simulink model "r2_b16a4x512f"  (R2012b)
settings: Solver=VariableStepDiscrete  SolverMode=SingleTasking  StartTime=0.0  StopTime=1  RelTol=1e-3
undefined symbols (not defined in the file): fft_stages, n_bits_ants, n_bits_xengs
libraries: xbsIndex_r4 x27410, casper_library_misc x230, xbsReplacements_r4 x24, casper_library_delays x8, xps_library x5, casper_library_communications x4
(part 116 of 229)

== system r2_b16a4x512f/sys2/xeng/baseline_tap7/dual_pol_cmac ==
  a1 : Inport
  a2 : Inport  Port=2
  acc_in : Inport  Port=3
  sync : Inport  Port=4
  valid_in : Inport  Port=5
  Concat : xbsIndex_r4/Concat  num_inputs=4  dbl_ovrd=off  block_type=concat
      settings: block_version=9.2.01
  Constant1 : xbsIndex_r4/Constant  const=0  gui_display_data_type=Fixed-point  arith_type=Unsigned  n_bits=1  bin_pt=0  preci_type=Single  exp_width=8  frac_width=24  explicit_period=on  period=1  equ=P=C  opselect=C  inp2=PCIN>>17  opr=+  inp1=P  carry=CIN  dbl_ovrd=off  block_type=constant
      settings: block_version=9.2.01
  Constant2 : xbsIndex_r4/Constant  const=0  gui_display_data_type=Fixed-point  arith_type=Unsigned  n_bits=1  bin_pt=0  preci_type=Single  exp_width=8  frac_width=24  explicit_period=on  period=1  equ=P=C  opselect=C  inp2=PCIN>>17  opr=+  inp1=P  carry=CIN  dbl_ovrd=off  block_type=constant
      settings: block_version=9.2.01
  Constant4 : xbsIndex_r4/Constant  const=0  gui_display_data_type=Fixed-point  arith_type=Unsigned  n_bits=1  bin_pt=0  preci_type=Single  exp_width=8  frac_width=24  explicit_period=on  period=1  equ=P=C  opselect=C  inp2=PCIN>>17  opr=+  inp1=P  carry=CIN  dbl_ovrd=off  block_type=constant
      settings: block_version=9.2.01
  Slice{,1,6,10} (4 alike) : xbsIndex_r4/Slice  nbits=2*n_bits  boolean_output=off  mode=Upper Bit Location + Width  bit1=0  base1=MSB of Input  bit0=0  base0=LSB of Input  dbl_ovrd=off  block_type=slice
      Slice settings: infoedit="Extracts a given range of bits from each input sample and presents it at the output.  The output type is ordinarily unsigned with binary point at zero, but can be Boolean when the slice is one bit wide.<P><P>Hardware notes: In hardware this block costs nothing."  block_version=9.2.01
      Slice1 settings: infoedit="Extracts a given range of bits from each input sample and presents it at the output.  The output type is ordinarily unsigned with binary point at zero, but can be Boolean when the slice is one bit wide.<P><P>Hardware notes: In hardware this block costs nothing."  block_version=9.2.01
      Slice10 settings: block_version=9.2.01
      Slice6 settings: infoedit="Extracts a given range of bits from each input sample and presents it at the output.  The output type is ordinarily unsigned with binary point at zero, but can be Boolean when the slice is one bit wide.<P><P>Hardware notes: In hardware this block costs nothing."  block_version=9.2.01
  Slice11 : xbsIndex_r4/Slice  nbits=2*n_bits_out  boolean_output=off  mode=Upper Bit Location + Width  bit1=-6*n_bits_out  base1=MSB of Input  bit0=0  base0=LSB of Input  dbl_ovrd=off  block_type=slice
      settings: infoedit="Extracts a given range of bits from each input sample and presents it at the output.  The output type is ordinarily unsigned with binary point at zero, but can be Boolean when the slice is one bit wide.<P><P>Hardware notes: In hardware this block costs nothing."  block_version=9.2.01
  Slice2 : xbsIndex_r4/Slice  nbits=2*n_bits_out  boolean_output=off  mode=Upper Bit Location + Width  bit1=0  base1=MSB of Input  bit0=0  base0=LSB of Input  dbl_ovrd=off  block_type=slice
      settings: infoedit="Extracts a given range of bits from each input sample and presents it at the output.  The output type is ordinarily unsigned with binary point at zero, but can be Boolean when the slice is one bit wide.<P><P>Hardware notes: In hardware this block costs nothing."  block_version=9.2.01
  Slice{3..4,7,9} (4 alike) : xbsIndex_r4/Slice  nbits=2*n_bits  boolean_output=off  mode=Upper Bit Location + Width  bit1=-2*n_bits  base1=MSB of Input  bit0=0  base0=LSB of Input  dbl_ovrd=off  block_type=slice
      Slice3 settings: infoedit="Extracts a given range of bits from each input sample and presents it at the output.  The output type is ordinarily unsigned with binary point at zero, but can be Boolean when the slice is one bit wide.<P><P>Hardware notes: In hardware this block costs nothing."  block_version=9.2.01
      Slice4 settings: infoedit="Extracts a given range of bits from each input sample and presents it at the output.  The output type is ordinarily unsigned with binary point at zero, but can be Boolean when the slice is one bit wide.<P><P>Hardware notes: In hardware this block costs nothing."  block_version=9.2.01
      Slice7 settings: infoedit="Extracts a given range of bits from each input sample and presents it at the output.  The output type is ordinarily unsigned with binary point at zero, but can be Boolean when the slice is one bit wide.<P><P>Hardware notes: In hardware this block costs nothing."  block_version=9.2.01
      Slice9 settings: block_version=9.2.01
  Slice5 : xbsIndex_r4/Slice  nbits=2*n_bits_out  boolean_output=off  mode=Upper Bit Location + Width  bit1=-2*n_bits_out  base1=MSB of Input  bit0=0  base0=LSB of Input  dbl_ovrd=off  block_type=slice
      settings: infoedit="Extracts a given range of bits from each input sample and presents it at the output.  The output type is ordinarily unsigned with binary point at zero, but can be Boolean when the slice is one bit wide.<P><P>Hardware notes: In hardware this block costs nothing."  block_version=9.2.01
  Slice8 : xbsIndex_r4/Slice  nbits=2*n_bits_out  boolean_output=off  mode=Upper Bit Location + Width  bit1=-4*n_bits_out  base1=MSB of Input  bit0=0  base0=LSB of Input  dbl_ovrd=off  block_type=slice
      settings: infoedit="Extracts a given range of bits from each input sample and presents it at the output.  The output type is ordinarily unsigned with binary point at zero, but can be Boolean when the slice is one bit wide.<P><P>Hardware notes: In hardware this block costs nothing."  block_version=9.2.01
  Terminator : Terminator
  Terminator1 : Terminator
  Terminator2 : Terminator
  cmac1 : Subsystem  Tag=cmac  AncestorBlock=casper_library_correlator/cmac  mask(cmac){acc_len=256, n_bits_a=8, bin_pt_a=7, n_bits_b=8, bin_pt_b=7, quantization=Truncate, overflow=Wrap, mult_latency=4, add_latency=3, in_latency=0, conv_latency=0, multiplier_implementation=embedded multiplier core}
      mask prompts: acc_len "Number of Accumulations"; n_bits_a "Number of bits 'a'"; bin_pt_a "Binary point 'a'"; n_bits_b "Number of bits 'b'"; bin_pt_b "Binary point 'b'"; quantization "Quantisation"; mult_latency "Multiplier Latency"; add_latency "Adder Latency"; in_latency "Input Latency"; conv_latency "Convert Latency"; multiplier_implementation "Multiplier Implementation"
      mask help: A complex multiply-accumulate block. Full precision.
      mask init: same as r2_b16a4x512f/sys0/xeng/auto_tap/dual_pol_cmac/cmac1
      mask TypeOptions quantization: Truncate | Round  (unbiased: +/- Inf) | Round  (unbiased: Even Values)
      mask TypeOptions overflow: Wrap | Saturate | Flag as error
      mask TypeOptions multiplier_implementation: behavioral HDL | standard core | embedded multiplier core
  cmac2 : Subsystem  Tag=cmac  AncestorBlock=casper_library_correlator/cmac  mask(cmac){acc_len=256, n_bits_a=8, bin_pt_a=7, n_bits_b=8, bin_pt_b=7, quantization=Truncate, overflow=Wrap, mult_latency=4, add_latency=3, in_latency=0, conv_latency=0, multiplier_implementation=embedded multiplier core}
      mask prompts: acc_len "Number of Accumulations"; n_bits_a "Number of bits 'a'"; bin_pt_a "Binary point 'a'"; n_bits_b "Number of bits 'b'"; bin_pt_b "Binary point 'b'"; quantization "Quantisation"; mult_latency "Multiplier Latency"; add_latency "Adder Latency"; in_latency "Input Latency"; conv_latency "Convert Latency"; multiplier_implementation "Multiplier Implementation"
      mask help: A complex multiply-accumulate block. Full precision.
      mask init: same as r2_b16a4x512f/sys0/xeng/auto_tap/dual_pol_cmac/cmac1
      mask TypeOptions quantization: Truncate | Round  (unbiased: +/- Inf) | Round  (unbiased: Even Values)
      mask TypeOptions overflow: Wrap | Saturate | Flag as error
      mask TypeOptions multiplier_implementation: behavioral HDL | standard core | embedded multiplier core
  cmac3 : Subsystem  Tag=cmac  AncestorBlock=casper_library_correlator/cmac  mask(cmac){acc_len=256, n_bits_a=8, bin_pt_a=7, n_bits_b=8, bin_pt_b=7, quantization=Truncate, overflow=Wrap, mult_latency=4, add_latency=3, in_latency=0, conv_latency=0, multiplier_implementation=embedded multiplier core}
      mask prompts: acc_len "Number of Accumulations"; n_bits_a "Number of bits 'a'"; bin_pt_a "Binary point 'a'"; n_bits_b "Number of bits 'b'"; bin_pt_b "Binary point 'b'"; quantization "Quantisation"; mult_latency "Multiplier Latency"; add_latency "Adder Latency"; in_latency "Input Latency"; conv_latency "Convert Latency"; multiplier_implementation "Multiplier Implementation"
      mask help: A complex multiply-accumulate block. Full precision.
      mask init: same as r2_b16a4x512f/sys0/xeng/auto_tap/dual_pol_cmac/cmac1
      mask TypeOptions quantization: Truncate | Round  (unbiased: +/- Inf) | Round  (unbiased: Even Values)
      mask TypeOptions overflow: Wrap | Saturate | Flag as error
      mask TypeOptions multiplier_implementation: behavioral HDL | standard core | embedded multiplier core
  cmac4 : Subsystem  Tag=cmac  AncestorBlock=casper_library_correlator/cmac  mask(cmac){acc_len=256, n_bits_a=8, bin_pt_a=7, n_bits_b=8, bin_pt_b=7, quantization=Truncate, overflow=Wrap, mult_latency=4, add_latency=3, in_latency=0, conv_latency=0, multiplier_implementation=embedded multiplier core}
      mask prompts: acc_len "Number of Accumulations"; n_bits_a "Number of bits 'a'"; bin_pt_a "Binary point 'a'"; n_bits_b "Number of bits 'b'"; bin_pt_b "Binary point 'b'"; quantization "Quantisation"; mult_latency "Multiplier Latency"; add_latency "Adder Latency"; in_latency "Input Latency"; conv_latency "Convert Latency"; multiplier_implementation "Multiplier Implementation"
      mask help: A complex multiply-accumulate block. Full precision.
      mask init: same as r2_b16a4x512f/sys0/xeng/auto_tap/dual_pol_cmac/cmac1
      mask TypeOptions quantization: Truncate | Round  (unbiased: +/- Inf) | Round  (unbiased: Even Values)
      mask TypeOptions overflow: Wrap | Saturate | Flag as error
      mask TypeOptions multiplier_implementation: behavioral HDL | standard core | embedded multiplier core
  acc_out : Outport
  valid_out : Outport  Port=2
  wires:
  acc_in/1 -> Slice2/1, Slice5/1, Slice8/1, Slice11/1
  a2/1 -> Slice10/1, Slice7/1, Slice4/1, Slice1/1
  a1/1 -> Slice9/1, Slice6/1, Slice3/1, Slice/1
  cmac4/1(acc_out) -> Concat/4
  cmac3/1(acc_out) -> Concat/3
  cmac2/1(acc_out) -> Concat/2
  cmac1/1(acc_out) -> Concat/1
  cmac4/2(valid_out) -> valid_out/1
  cmac3/2(valid_out) -> Terminator2/1
  cmac2/2(valid_out) -> Terminator1/1
  sync/1 -> cmac4/4(sync), cmac3/4(sync), cmac2/4(sync), cmac1/4(sync)
  Slice11/1 -> cmac4/3(acc_in)
  Slice10/1 -> cmac4/2(c+di)
  Slice9/1 -> cmac4/1(a+bi)
  Constant4/1 -> cmac3/5(valid_in)
  Slice8/1 -> cmac3/3(acc_in)
  Slice7/1 -> cmac3/2(c+di)
  Slice6/1 -> cmac3/1(a+bi)
  Constant1/1 -> cmac2/5(valid_in)
  cmac1/2(valid_out) -> Terminator/1
  valid_in/1 -> cmac4/5(valid_in)
  Concat/1 -> acc_out/1
  Slice5/1 -> cmac2/3(acc_in)
  Slice4/1 -> cmac2/2(c+di)
  Slice3/1 -> cmac2/1(a+bi)
  Slice2/1 -> cmac1/3(acc_in)
  Slice1/1 -> cmac1/2(c+di)
  Slice/1 -> cmac1/1(a+bi)
  Constant2/1 -> cmac1/5(valid_in)

== system r2_b16a4x512f/sys2/xeng/baseline_tap8/delay ==
  din : Inport
  constant : xbsIndex_r4/Constant  const=1  gui_display_data_type=Fixed-point  arith_type=Boolean  n_bits=16  bin_pt=14  preci_type=Single  exp_width=8  frac_width=24  explicit_period=on  period=1  equ=P=C  opselect=C  inp2=PCIN>>17  opr=+  inp1=P  carry=CIN  dbl_ovrd=off  block_type=constant
  counter : xbsIndex_r4/Counter  cnt_type=Count Limited  cnt_to=DelayLen - bram_latency - 1  operation=Up  start_count=0  cnt_by_val=1  arith_type=Unsigned  n_bits=8  bin_pt=0  load_pin=off  rst=off  en=off  explicit_period=on  period=1  dbl_ovrd=off  use_behavioral_HDL=off  implementation=Fabric  use_rpm=off  block_type=counter
  ram : xbsIndex_r4/Single Port RAM  depth=256  initVector=0  distributed_mem=Block RAM  write_mode=Read Before Write  rst=off  init_reg=0  en=off  latency=bram_latency  dbl_ovrd=off  optimize=Area  block_type=spram
  dout : Outport
  wires:
  counter/1 -> ram/1
  din/1 -> ram/2
  constant/1 -> ram/3
  ram/1 -> dout/1

== system r2_b16a4x512f/sys2/xeng/baseline_tap8/dual_pol_cmac ==
  a1 : Inport
  a2 : Inport  Port=2
  acc_in : Inport  Port=3
  sync : Inport  Port=4
  valid_in : Inport  Port=5
  Concat : xbsIndex_r4/Concat  num_inputs=4  dbl_ovrd=off  block_type=concat
      settings: block_version=9.2.01
  Constant1 : xbsIndex_r4/Constant  const=0  gui_display_data_type=Fixed-point  arith_type=Unsigned  n_bits=1  bin_pt=0  preci_type=Single  exp_width=8  frac_width=24  explicit_period=on  period=1  equ=P=C  opselect=C  inp2=PCIN>>17  opr=+  inp1=P  carry=CIN  dbl_ovrd=off  block_type=constant
      settings: block_version=9.2.01
  Constant2 : xbsIndex_r4/Constant  const=0  gui_display_data_type=Fixed-point  arith_type=Unsigned  n_bits=1  bin_pt=0  preci_type=Single  exp_width=8  frac_width=24  explicit_period=on  period=1  equ=P=C  opselect=C  inp2=PCIN>>17  opr=+  inp1=P  carry=CIN  dbl_ovrd=off  block_type=constant
      settings: block_version=9.2.01
  Constant4 : xbsIndex_r4/Constant  const=0  gui_display_data_type=Fixed-point  arith_type=Unsigned  n_bits=1  bin_pt=0  preci_type=Single  exp_width=8  frac_width=24  explicit_period=on  period=1  equ=P=C  opselect=C  inp2=PCIN>>17  opr=+  inp1=P  carry=CIN  dbl_ovrd=off  block_type=constant
      settings: block_version=9.2.01
  Slice{,1,6,10} (4 alike) : xbsIndex_r4/Slice  nbits=2*n_bits  boolean_output=off  mode=Upper Bit Location + Width  bit1=0  base1=MSB of Input  bit0=0  base0=LSB of Input  dbl_ovrd=off  block_type=slice
      Slice settings: infoedit="Extracts a given range of bits from each input sample and presents it at the output.  The output type is ordinarily unsigned with binary point at zero, but can be Boolean when the slice is one bit wide.<P><P>Hardware notes: In hardware this block costs nothing."  block_version=9.2.01
      Slice1 settings: infoedit="Extracts a given range of bits from each input sample and presents it at the output.  The output type is ordinarily unsigned with binary point at zero, but can be Boolean when the slice is one bit wide.<P><P>Hardware notes: In hardware this block costs nothing."  block_version=9.2.01
      Slice10 settings: block_version=9.2.01
      Slice6 settings: infoedit="Extracts a given range of bits from each input sample and presents it at the output.  The output type is ordinarily unsigned with binary point at zero, but can be Boolean when the slice is one bit wide.<P><P>Hardware notes: In hardware this block costs nothing."  block_version=9.2.01
  Slice11 : xbsIndex_r4/Slice  nbits=2*n_bits_out  boolean_output=off  mode=Upper Bit Location + Width  bit1=-6*n_bits_out  base1=MSB of Input  bit0=0  base0=LSB of Input  dbl_ovrd=off  block_type=slice
      settings: infoedit="Extracts a given range of bits from each input sample and presents it at the output.  The output type is ordinarily unsigned with binary point at zero, but can be Boolean when the slice is one bit wide.<P><P>Hardware notes: In hardware this block costs nothing."  block_version=9.2.01
  Slice2 : xbsIndex_r4/Slice  nbits=2*n_bits_out  boolean_output=off  mode=Upper Bit Location + Width  bit1=0  base1=MSB of Input  bit0=0  base0=LSB of Input  dbl_ovrd=off  block_type=slice
      settings: infoedit="Extracts a given range of bits from each input sample and presents it at the output.  The output type is ordinarily unsigned with binary point at zero, but can be Boolean when the slice is one bit wide.<P><P>Hardware notes: In hardware this block costs nothing."  block_version=9.2.01
  Slice{3..4,7,9} (4 alike) : xbsIndex_r4/Slice  nbits=2*n_bits  boolean_output=off  mode=Upper Bit Location + Width  bit1=-2*n_bits  base1=MSB of Input  bit0=0  base0=LSB of Input  dbl_ovrd=off  block_type=slice
      Slice3 settings: infoedit="Extracts a given range of bits from each input sample and presents it at the output.  The output type is ordinarily unsigned with binary point at zero, but can be Boolean when the slice is one bit wide.<P><P>Hardware notes: In hardware this block costs nothing."  block_version=9.2.01
      Slice4 settings: infoedit="Extracts a given range of bits from each input sample and presents it at the output.  The output type is ordinarily unsigned with binary point at zero, but can be Boolean when the slice is one bit wide.<P><P>Hardware notes: In hardware this block costs nothing."  block_version=9.2.01
      Slice7 settings: infoedit="Extracts a given range of bits from each input sample and presents it at the output.  The output type is ordinarily unsigned with binary point at zero, but can be Boolean when the slice is one bit wide.<P><P>Hardware notes: In hardware this block costs nothing."  block_version=9.2.01
      Slice9 settings: block_version=9.2.01
  Slice5 : xbsIndex_r4/Slice  nbits=2*n_bits_out  boolean_output=off  mode=Upper Bit Location + Width  bit1=-2*n_bits_out  base1=MSB of Input  bit0=0  base0=LSB of Input  dbl_ovrd=off  block_type=slice
      settings: infoedit="Extracts a given range of bits from each input sample and presents it at the output.  The output type is ordinarily unsigned with binary point at zero, but can be Boolean when the slice is one bit wide.<P><P>Hardware notes: In hardware this block costs nothing."  block_version=9.2.01
  Slice8 : xbsIndex_r4/Slice  nbits=2*n_bits_out  boolean_output=off  mode=Upper Bit Location + Width  bit1=-4*n_bits_out  base1=MSB of Input  bit0=0  base0=LSB of Input  dbl_ovrd=off  block_type=slice
      settings: infoedit="Extracts a given range of bits from each input sample and presents it at the output.  The output type is ordinarily unsigned with binary point at zero, but can be Boolean when the slice is one bit wide.<P><P>Hardware notes: In hardware this block costs nothing."  block_version=9.2.01
  Terminator : Terminator
  Terminator1 : Terminator
  Terminator2 : Terminator
  cmac1 : Subsystem  Tag=cmac  AncestorBlock=casper_library_correlator/cmac  mask(cmac){acc_len=256, n_bits_a=8, bin_pt_a=7, n_bits_b=8, bin_pt_b=7, quantization=Truncate, overflow=Wrap, mult_latency=4, add_latency=3, in_latency=0, conv_latency=0, multiplier_implementation=embedded multiplier core}
      mask prompts: acc_len "Number of Accumulations"; n_bits_a "Number of bits 'a'"; bin_pt_a "Binary point 'a'"; n_bits_b "Number of bits 'b'"; bin_pt_b "Binary point 'b'"; quantization "Quantisation"; mult_latency "Multiplier Latency"; add_latency "Adder Latency"; in_latency "Input Latency"; conv_latency "Convert Latency"; multiplier_implementation "Multiplier Implementation"
      mask help: A complex multiply-accumulate block. Full precision.
      mask init: same as r2_b16a4x512f/sys0/xeng/auto_tap/dual_pol_cmac/cmac1
      mask TypeOptions quantization: Truncate | Round  (unbiased: +/- Inf) | Round  (unbiased: Even Values)
      mask TypeOptions overflow: Wrap | Saturate | Flag as error
      mask TypeOptions multiplier_implementation: behavioral HDL | standard core | embedded multiplier core
  cmac2 : Subsystem  Tag=cmac  AncestorBlock=casper_library_correlator/cmac  mask(cmac){acc_len=256, n_bits_a=8, bin_pt_a=7, n_bits_b=8, bin_pt_b=7, quantization=Truncate, overflow=Wrap, mult_latency=4, add_latency=3, in_latency=0, conv_latency=0, multiplier_implementation=embedded multiplier core}
      mask prompts: acc_len "Number of Accumulations"; n_bits_a "Number of bits 'a'"; bin_pt_a "Binary point 'a'"; n_bits_b "Number of bits 'b'"; bin_pt_b "Binary point 'b'"; quantization "Quantisation"; mult_latency "Multiplier Latency"; add_latency "Adder Latency"; in_latency "Input Latency"; conv_latency "Convert Latency"; multiplier_implementation "Multiplier Implementation"
      mask help: A complex multiply-accumulate block. Full precision.
      mask init: same as r2_b16a4x512f/sys0/xeng/auto_tap/dual_pol_cmac/cmac1
      mask TypeOptions quantization: Truncate | Round  (unbiased: +/- Inf) | Round  (unbiased: Even Values)
      mask TypeOptions overflow: Wrap | Saturate | Flag as error
      mask TypeOptions multiplier_implementation: behavioral HDL | standard core | embedded multiplier core
  cmac3 : Subsystem  Tag=cmac  AncestorBlock=casper_library_correlator/cmac  mask(cmac){acc_len=256, n_bits_a=8, bin_pt_a=7, n_bits_b=8, bin_pt_b=7, quantization=Truncate, overflow=Wrap, mult_latency=4, add_latency=3, in_latency=0, conv_latency=0, multiplier_implementation=embedded multiplier core}
      mask prompts: acc_len "Number of Accumulations"; n_bits_a "Number of bits 'a'"; bin_pt_a "Binary point 'a'"; n_bits_b "Number of bits 'b'"; bin_pt_b "Binary point 'b'"; quantization "Quantisation"; mult_latency "Multiplier Latency"; add_latency "Adder Latency"; in_latency "Input Latency"; conv_latency "Convert Latency"; multiplier_implementation "Multiplier Implementation"
      mask help: A complex multiply-accumulate block. Full precision.
      mask init: same as r2_b16a4x512f/sys0/xeng/auto_tap/dual_pol_cmac/cmac1
      mask TypeOptions quantization: Truncate | Round  (unbiased: +/- Inf) | Round  (unbiased: Even Values)
      mask TypeOptions overflow: Wrap | Saturate | Flag as error
      mask TypeOptions multiplier_implementation: behavioral HDL | standard core | embedded multiplier core
  cmac4 : Subsystem  Tag=cmac  AncestorBlock=casper_library_correlator/cmac  mask(cmac){acc_len=256, n_bits_a=8, bin_pt_a=7, n_bits_b=8, bin_pt_b=7, quantization=Truncate, overflow=Wrap, mult_latency=4, add_latency=3, in_latency=0, conv_latency=0, multiplier_implementation=embedded multiplier core}
      mask prompts: acc_len "Number of Accumulations"; n_bits_a "Number of bits 'a'"; bin_pt_a "Binary point 'a'"; n_bits_b "Number of bits 'b'"; bin_pt_b "Binary point 'b'"; quantization "Quantisation"; mult_latency "Multiplier Latency"; add_latency "Adder Latency"; in_latency "Input Latency"; conv_latency "Convert Latency"; multiplier_implementation "Multiplier Implementation"
      mask help: A complex multiply-accumulate block. Full precision.
      mask init: same as r2_b16a4x512f/sys0/xeng/auto_tap/dual_pol_cmac/cmac1
      mask TypeOptions quantization: Truncate | Round  (unbiased: +/- Inf) | Round  (unbiased: Even Values)
      mask TypeOptions overflow: Wrap | Saturate | Flag as error
      mask TypeOptions multiplier_implementation: behavioral HDL | standard core | embedded multiplier core
  acc_out : Outport
  valid_out : Outport  Port=2
  wires:
  acc_in/1 -> Slice2/1, Slice5/1, Slice8/1, Slice11/1
  a2/1 -> Slice10/1, Slice7/1, Slice4/1, Slice1/1
  a1/1 -> Slice9/1, Slice6/1, Slice3/1, Slice/1
  cmac4/1(acc_out) -> Concat/4
  cmac3/1(acc_out) -> Concat/3
  cmac2/1(acc_out) -> Concat/2
  cmac1/1(acc_out) -> Concat/1
  cmac4/2(valid_out) -> valid_out/1
  cmac3/2(valid_out) -> Terminator2/1
  cmac2/2(valid_out) -> Terminator1/1
  sync/1 -> cmac4/4(sync), cmac3/4(sync), cmac2/4(sync), cmac1/4(sync)
  Slice11/1 -> cmac4/3(acc_in)
  Slice10/1 -> cmac4/2(c+di)
  Slice9/1 -> cmac4/1(a+bi)
  Constant4/1 -> cmac3/5(valid_in)
  Slice8/1 -> cmac3/3(acc_in)
  Slice7/1 -> cmac3/2(c+di)
  Slice6/1 -> cmac3/1(a+bi)
  Constant1/1 -> cmac2/5(valid_in)
  cmac1/2(valid_out) -> Terminator/1
  valid_in/1 -> cmac4/5(valid_in)
  Concat/1 -> acc_out/1
  Slice5/1 -> cmac2/3(acc_in)
  Slice4/1 -> cmac2/2(c+di)
  Slice3/1 -> cmac2/1(a+bi)
  Slice2/1 -> cmac1/3(acc_in)
  Slice1/1 -> cmac1/2(c+di)
  Slice/1 -> cmac1/1(a+bi)
  Constant2/1 -> cmac1/5(valid_in)

== system r2_b16a4x512f/sys2/xeng/xeng_descramble/read_ctrl ==
  start : Inport
  Constant1 : xbsIndex_r4/Constant  const=ship_el_cnt  gui_display_data_type=Fixed-point  arith_type=Unsigned  n_bits=ceil(log2(ship_el_cnt+1))  bin_pt=0  preci_type=Single  exp_width=8  frac_width=24  explicit_period=on  period=1  equ=P=C  opselect=C  inp2=PCIN>>17  opr=+  inp1=P  carry=CIN  dbl_ovrd=off  block_type=constant
      settings: block_version=9.2.01
  Constant2 : xbsIndex_r4/Constant  const=ship_el_del  gui_display_data_type=Fixed-point  arith_type=Unsigned  n_bits=ship_el_del_bits  bin_pt=0  preci_type=Single  exp_width=8  frac_width=24  explicit_period=on  period=1  equ=P=C  opselect=C  inp2=PCIN>>17  opr=+  inp1=P  carry=CIN  dbl_ovrd=off  block_type=constant
      settings: block_version=9.2.01
  Gateway Out{1..2,4..8} (7 alike) : xbsIndex_r4/Gateway Out  inherit_from_input=off  hdl_port=off  timing_constraint=None  locs_specified=off  LOCs={}  UseAsDAC=off  DACChannel='1'  block_type=gatewayout
      settings: infoedit="Gateway out block.  Converts Xilinx fixed point inputs into ouputs of type Simulink integer, double, or fixed point.<P><P>Hardware notes:  In hardware these blocks become top level output ports or are discarded, depending on how they are configured."  xl_area=[0, 0, 0, 0, 0, 0, 0]  block_version=10.1.3
  Inverter3 : xbsIndex_r4/Inverter  en=off  latency=0  dbl_ovrd=off  block_type=inv
      settings: xl_area=[0, 0, 0, 0, 0, 0, 0]  block_version=9.2.01
  Logical1 : xbsIndex_r4/Logical  logical_function=AND  inputs=2  en=off  latency=0  precision=Full  arith_type=Unsigned  n_bits=8  bin_pt=2  align_bp=on  dbl_ovrd=off  block_type=logical
      settings: xl_area=[0, 0, 0, 0, 0, 0, 0]  block_version=9.2.01
  Logical7 : xbsIndex_r4/Logical  logical_function=OR  inputs=2  en=off  latency=0  precision=Full  arith_type=Unsigned  n_bits=8  bin_pt=2  align_bp=on  dbl_ovrd=off  block_type=logical
      settings: xl_area=[0, 0, 0, 0, 0, 0, 0]  block_version=9.2.01
  Register : xbsIndex_r4/Register  init=0  rst=on  en=on  dbl_ovrd=off  block_type=register
  Relational1 : xbsIndex_r4/Relational  mode=a<=b  en=off  latency=0  dbl_ovrd=off  block_type=relational
      settings: xl_area=[0, 0, 0, 0, 0, 0, 0]  block_version=9.2.01
  Relational3 : xbsIndex_r4/Relational  mode=a<=b  en=off  latency=0  dbl_ovrd=off  block_type=relational
      settings: xl_area=[0, 0, 0, 0, 0, 0, 0]  block_version=9.2.01
  Scope1 : Scope  NumInputPorts=7
      settings: YMin=0~0~0~0~0~0~0  YMax=1~20~1~1~9~1~9
  element : xbsIndex_r4/Counter  cnt_type=Free Running  cnt_to=demux_factor*num_elements+1  operation=Up  start_count=0  cnt_by_val=1  arith_type=Unsigned  n_bits=ceil(log2(ship_el_cnt+1))  bin_pt=0  load_pin=off  rst=on  en=on  explicit_period=off  period=1  dbl_ovrd=off  use_behavioral_HDL=off  implementation=Fabric  use_rpm=on  block_type=counter
      settings: xl_area=[0, 0, 0, 0, 0, 0, 0]  block_version=9.2.01
  ship_element_delay : xbsIndex_r4/Counter  cnt_type=Free Running  cnt_to=1  operation=Up  start_count=0  cnt_by_val=1  arith_type=Unsigned  n_bits=ship_el_del_bits  bin_pt=0  load_pin=off  rst=on  en=off  explicit_period=off  period=1  dbl_ovrd=off  use_behavioral_HDL=off  implementation=Fabric  use_rpm=on  block_type=counter
      settings: xl_area=[0, 0, 0, 0, 0, 0, 0]  block_version=9.2.01
  read_addr : Outport
  enable : Outport  Port=2
  wires:
  Relational3/1 -> Register/3, Register/1
  Inverter3/1 -> Logical1/2
  Register/1 -> Inverter3/1
  Logical1/1 -> element/2, Gateway Out1/1, enable/1, Gateway Out4/1
  Gateway Out2/1 -> Scope1/7
  Gateway Out1/1 -> Scope1/6
  Gateway Out8/1 -> Scope1/3
  Gateway Out6/1 -> Scope1/2
  Gateway Out5/1 -> Scope1/1
  Gateway Out4/1 -> Scope1/4
  Gateway Out7/1 -> Scope1/5
  Relational1/1 -> Logical1/1, Logical7/2, Gateway Out8/1
  Logical7/1 -> ship_element_delay/1
  ship_element_delay/1 -> Gateway Out6/1, Relational1/2
  Constant2/1 -> Relational1/1
  Constant1/1 -> Relational3/1
  element/1 -> Gateway Out2/1, read_addr/1, Relational3/2, Gateway Out7/1
  start/1 -> Register/2, element/1, Gateway Out5/1, Logical7/1

== system r2_b16a4x512f/sys2/xeng/xeng_descramble/write_ctrl ==
  note: Lock onto start of new
      | valid window if previous
      | window was invalid
  note: negedge delay to
      | accomodate
      | a valid window followed
      | by an invalid window
  note: Flip this ordering to correct for
      | AxBx,AyBy,AyBx,AxBy ->AxBx,AyBy,AxBy,AyBx
  sync : Inport
  data_in : Inport  Port=2
  xeng_valid : Inport  Port=3
  window_valid : Inport  Port=4
  AddSub : xbsIndex_r4/AddSub  mode=Subtraction  use_carryin=off  use_carryout=off  en=off  latency=0  precision=Full  arith_type=Unsigned  n_bits=8  bin_pt=2  quantization=Truncate  overflow=Wrap  dbl_ovrd=off  use_behavioral_HDL=on  hw_selection=Fabric  pipelined=off  use_rpm=on  block_type=addsub
      settings: xl_area=[0, 0, 0, 0, 0, 0, 0]  block_version=9.2.01
  Constant : xbsIndex_r4/Constant  const=num_taps-1  gui_display_data_type=Fixed-point  arith_type=Unsigned  n_bits=taps_bits  bin_pt=0  preci_type=Single  exp_width=8  frac_width=24  explicit_period=on  period=1  equ=P=C  opselect=C  inp2=PCIN>>17  opr=+  inp1=P  carry=CIN  dbl_ovrd=off  block_type=constant
      settings: block_version=9.2.01
  Constant3 : xbsIndex_r4/Constant  const=ceil(num_validins*3/4)  gui_display_data_type=Fixed-point  arith_type=Unsigned  n_bits=validin_bits  bin_pt=0  preci_type=Single  exp_width=8  frac_width=24  explicit_period=on  period=1  equ=P=C  opselect=C  inp2=PCIN>>17  opr=+  inp1=P  carry=CIN  dbl_ovrd=off  block_type=constant
      settings: block_version=9.2.01
  Constant5 : xbsIndex_r4/Constant  const=0  gui_display_data_type=Fixed-point  arith_type=Unsigned  n_bits=taps_bits  bin_pt=0  preci_type=Single  exp_width=8  frac_width=24  explicit_period=on  period=1  equ=P=C  opselect=C  inp2=PCIN>>17  opr=+  inp1=P  carry=CIN  dbl_ovrd=off  block_type=constant
      settings: block_version=9.2.01
  Constant7 : xbsIndex_r4/Constant  const=num_taps-1  gui_display_data_type=Fixed-point  arith_type=Unsigned  n_bits=taps_bits  bin_pt=0  preci_type=Single  exp_width=8  frac_width=24  explicit_period=on  period=1  equ=P=C  opselect=C  inp2=PCIN>>17  opr=+  inp1=P  carry=CIN  dbl_ovrd=off  block_type=constant
      settings: block_version=9.2.01
  Convert : xbsIndex_r4/Convert  gui_display_data_type=Fixed-point  arith_type=Unsigned  n_bits=taps_bits+1  bin_pt=0  float_type=Single  exp_bits=8  fraction_bits=24  quantization=Truncate  overflow=Wrap  en=off  latency=0  dbl_ovrd=off  pipeline=off  block_type=convert
      settings: xl_area=[0, 0, 0, 0, 0, 0, 0]  block_version=9.2.01
  Counter2 : xbsIndex_r4/Counter  cnt_type=Count Limited  cnt_to=num_elements-1  operation=Up  start_count=pivot_pnt  cnt_by_val=1  arith_type=Unsigned  n_bits=ceil(log2(num_elements))  bin_pt=0  load_pin=off  rst=on  en=on  explicit_period=off  period=1  dbl_ovrd=off  use_behavioral_HDL=off  implementation=Fabric  use_rpm=on  block_type=counter
      settings: xl_area=[0, 0, 0, 0, 0, 0, 0]  block_version=9.2.01
  Counter3 : xbsIndex_r4/Counter  cnt_type=Count Limited  cnt_to=pivot_pnt-1  operation=Up  start_count=0  cnt_by_val=1  arith_type=Unsigned  n_bits=ceil(log2(num_elements))  bin_pt=0  load_pin=off  rst=on  en=on  explicit_period=off  period=1  dbl_ovrd=off  use_behavioral_HDL=off  implementation=Fabric  use_rpm=on  block_type=counter
      settings: xl_area=[0, 0, 0, 0, 0, 0, 0]  block_version=9.2.01
  Delay{,1..6} (7 alike) : xbsIndex_r4/Delay  rst=off  infoeditControl=Selection of Reset will increase slice count due to use of real FFs and instead of SRLs  en=off  latency=1  dbl_ovrd=off  reg_retiming=on  block_type=delay
  Gateway Out{1..8} (8 alike) : xbsIndex_r4/Gateway Out  inherit_from_input=off  hdl_port=off  timing_constraint=None  locs_specified=off  LOCs={}  UseAsDAC=off  DACChannel='1'  block_type=gatewayout
      settings: infoedit="Gateway out block.  Converts Xilinx fixed point inputs into ouputs of type Simulink integer, double, or fixed point.<P><P>Hardware notes:  In hardware these blocks become top level output ports or are discarded, depending on how they are configured."  xl_area=[0, 0, 0, 0, 0, 0, 0]  block_version=10.1.3
  Inverter{,1..3} (4 alike) : xbsIndex_r4/Inverter  en=off  latency=0  dbl_ovrd=off  block_type=inv
      settings: xl_area=[0, 0, 0, 0, 0, 0, 0]  block_version=9.2.01
  Logical{,2..3,5,7} (5 alike) : xbsIndex_r4/Logical  logical_function=AND  inputs=2  en=off  latency=0  precision=Full  arith_type=Unsigned  n_bits=8  bin_pt=2  align_bp=on  dbl_ovrd=off  block_type=logical
      settings: xl_area=[0, 0, 0, 0, 0, 0, 0]  block_version=9.2.01
  Logical1 : xbsIndex_r4/Logical  logical_function=OR  inputs=2  en=off  latency=0  precision=Full  arith_type=Unsigned  n_bits=8  bin_pt=2  align_bp=on  dbl_ovrd=off  block_type=logical
      settings: xl_area=[0, 0, 0, 0, 0, 0, 0]  block_version=9.2.01
  Logical4 : xbsIndex_r4/Logical  logical_function=AND  inputs=3  en=off  latency=0  precision=Full  arith_type=Unsigned  n_bits=8  bin_pt=2  align_bp=on  dbl_ovrd=off  block_type=logical
      settings: xl_area=[0, 0, 0, 0, 0, 0, 0]  block_version=9.2.01
  Logical6 : xbsIndex_r4/Logical  logical_function=OR  inputs=2  en=off  latency=0  precision=Full  arith_type=Unsigned  n_bits=8  bin_pt=2  align_bp=on  dbl_ovrd=off  block_type=logical
      settings: xl_area=[0, 0, 0, 0, 0, 0, 0]  block_version=9.2.01
  Mux : xbsIndex_r4/Mux  inputs=2  en=off  latency=0  precision=Full  arith_type="Signed  (2's comp)"  n_bits=8  bin_pt=2  quantization=Truncate  overflow=Wrap  dbl_ovrd=off  block_type=mux
      settings: xl_area=[0, 0, 0, 0, 0, 0, 0]  block_version=9.2.01
  Relational : xbsIndex_r4/Relational  mode=a=b  en=off  latency=0  dbl_ovrd=off  block_type=relational
      settings: xl_area=[0, 0, 0, 0, 0, 0, 0]  block_version=9.2.01
  Relational1 : xbsIndex_r4/Relational  mode=a>=b  en=off  latency=1  dbl_ovrd=off  block_type=relational
      settings: xl_area=[0, 0, 0, 0, 0, 0, 0]  block_version=9.2.01
  Relational3 : xbsIndex_r4/Relational  mode=a=b  en=off  latency=1  dbl_ovrd=off  block_type=relational
      settings: xl_area=[0, 0, 0, 0, 0, 0, 0]  block_version=9.2.01
  Relational4 : xbsIndex_r4/Relational  mode=a=b  en=off  latency=1  dbl_ovrd=off  block_type=relational
      settings: xl_area=[0, 0, 0, 0, 0, 0, 0]  block_version=9.2.01
  element_number : xbsIndex_r4/Counter  cnt_type=Count Limited  cnt_to=num_validins-1  operation=Up  start_count=0  cnt_by_val=1  arith_type=Unsigned  n_bits=validin_bits  bin_pt=0  load_pin=off  rst=on  en=on  explicit_period=off  period=1  dbl_ovrd=off  use_behavioral_HDL=off  implementation=Fabric  use_rpm=on  block_type=counter
      settings: xl_area=[0, 0, 0, 0, 0, 0, 0]  block_version=9.2.01
  line_number : xbsIndex_r4/Counter  cnt_type=Count Limited  cnt_to=num_ants-1  operation=Up  start_count=0  cnt_by_val=1  arith_type=Unsigned  n_bits=ant_bits  bin_pt=0  load_pin=off  rst=on  en=on  explicit_period=off  period=1  dbl_ovrd=off  use_behavioral_HDL=off  implementation=Fabric  use_rpm=on  block_type=counter
      settings: xl_area=[0, 0, 0, 0, 0, 0, 0]  block_version=9.2.01
  negate{1..4} (4 alike) : xbsIndex_r4/Negate  precision=User Defined  arith_type="Signed  (2's comp)"  n_bits=n_bits_xeng_out  bin_pt=0  quantization=Truncate  overflow=Wrap  en=off  latency=0  dbl_ovrd=off  block_type=negate
      negate1 settings: block_version=11.4
      negate2 settings: AttributesFormatString=num_ants=8  block_version=11.4
      negate3 settings: block_version=11.4
      negate4 settings: block_version=11.4
  negedge_delay : Subsystem  AncestorBlock=casper_library_misc/negedge_delay  mask(negedge_delay){pulse_len=ceil(num_ants/2)*acc_len}
      mask prompts: pulse_len "Length of Pulse"
      mask help:
      | Extends a boolean signal to be high for the specified number of clocks after
      | the last high input (negative edge).
      |
      | Minimum length is 3.
      mask init:
      | bits = ceil(log2(pulse_len+1));
      | 
      | if pulse_len < 3,
      |     errordlg('Minimum length is 3.');
      | end
  posedge : casper_library_misc/edge_detect  edge=Rising  polarity=Active High  x_in=[0 0.08 0.08 0.16 0.16 0.24 0.24 0.32 0.32 0.4]  y_in="[-1 -1  1  1  1  1  1  1  1  1]"  x_out=[0.6 0.68 0.68 0.76 0.76 0.84 0.84 0.92 0.92 1]  y_out="[-1 -1  1  1 -1 -1 -1 -1 -1 -1]"
  posedge1 : casper_library_misc/edge_detect  edge=Rising  polarity=Active High  x_in=[0 0.08 0.08 0.16 0.16 0.24 0.24 0.32 0.32 0.4]  y_in="[-1 -1  1  1  1  1  1  1  1  1]"  x_out=[0.6 0.68 0.68 0.76 0.76 0.84 0.84 0.92 0.92 1]  y_out="[-1 -1  1  1 -1 -1 -1 -1 -1 -1]"
  remux : xbsIndex_r4/Concat  num_inputs=4  dbl_ovrd=off  block_type=concat
  repack{1..4} (4 alike) : casper_library_misc/ri_to_c
  sel_conj : xbsIndex_r4/Mux  inputs=2  en=off  latency=0  precision=Full  arith_type=Unsigned  n_bits=16  bin_pt=14  quantization=Truncate  overflow=Wrap  dbl_ovrd=off  block_type=mux
  slice1 : xbsIndex_r4/Slice  nbits=2*n_bits_xeng_out  boolean_output=off  mode=Lower Bit Location + Width  bit1=0  base1=MSB of Input  bit0=2*n_bits_xeng_out*3  base0=LSB of Input  dbl_ovrd=off  block_type=slice
  slice2 : xbsIndex_r4/Slice  nbits=2*n_bits_xeng_out  boolean_output=off  mode=Lower Bit Location + Width  bit1=0  base1=MSB of Input  bit0=4*n_bits_xeng_out  base0=LSB of Input  dbl_ovrd=off  block_type=slice
  slice3 : xbsIndex_r4/Slice  nbits=2*n_bits_xeng_out  boolean_output=off  mode=Lower Bit Location + Width  bit1=0  base1=MSB of Input  bit0=2*n_bits_xeng_out  base0=LSB of Input  dbl_ovrd=off  block_type=slice
  slice4 : xbsIndex_r4/Slice  nbits=2*n_bits_xeng_out  boolean_output=off  mode=Lower Bit Location + Width  bit1=0  base1=MSB of Input  bit0=0  base0=LSB of Input  dbl_ovrd=off  block_type=slice
  tap_number : xbsIndex_r4/Counter  cnt_type=Count Limited  cnt_to=num_taps-1  operation=Up  start_count=0  cnt_by_val=1  arith_type=Unsigned  n_bits=taps_bits  bin_pt=0  load_pin=off  rst=on  en=on  explicit_period=off  period=1  dbl_ovrd=off  use_behavioral_HDL=off  implementation=Fabric  use_rpm=on  block_type=counter
      settings: xl_area=[0, 0, 0, 0, 0, 0, 0]  block_version=9.2.01
  unpack{1..4} (4 alike) : casper_library_misc/c_to_ri  n_bits=n_bits_xeng_out  bin_pt=0
      settings: AttributesFormatString=25_0 r/i
  wr_ctl_debug : Scope  NumInputPorts=8
      settings: YMin=0~0~0~0~30~0~0~-5  YMax=1~1~1~1~39~40~40~5  SaveName=ScopeData5
  start_readout : Outport
  write_addr : Outport  Port=2
  data_out : Outport  Port=3
  enable : Outport  Port=4
  wires:
  Delay3/1 -> [data_in]
  data_in/1 -> Delay3/1
  Delay1/1 -> [valid_in]
  sync/1 -> Delay/1
  Logical1/1 -> [rst_in]
  xeng_valid/1 -> Logical2/2
  posedge/1 -> Logical1/2
  Delay/1 -> Logical1/1
  window_valid/1 -> negedge_delay/1(in), posedge/1
  Logical2/1 -> Delay1/1
  negedge_delay/1(out) -> Logical2/1
  [data_in] -> Delay6/1
  [last_triangle] -> sel_conj/1
  repack4/1 -> remux/3
  repack3/1 -> remux/4
  Delay6/1 -> sel_conj/2, slice1/1, slice2/1, slice3/1, slice4/1
  sel_conj/1 -> data_out/1
  remux/1 -> sel_conj/3
  slice1/1 -> unpack1/1
  unpack1/1 -> repack1/1
  unpack1/2 -> negate1/1
  negate1/1 -> repack1/2
  repack1/1 -> remux/1
  slice2/1 -> unpack2/1
  unpack2/1 -> repack2/1
  unpack2/2 -> negate2/1
  negate2/1 -> repack2/2
  repack2/1 -> remux/2
  slice3/1 -> unpack3/1
  unpack3/1 -> repack3/1
  unpack3/2 -> negate3/1
  negate3/1 -> repack3/2
  slice4/1 -> unpack4/1
  unpack4/1 -> repack4/1
  unpack4/2 -> negate4/1
  negate4/1 -> repack4/2
  Delay2/1 -> [pos_cnt]
  posedge1/1 -> start_readout/1
  Relational/1 -> Logical/1, Logical6/1
  [valid_in] -> Logical6/2
  [valid_in] -> Logical/2
  [valid_in] -> element_number/2
  Delay5/1 -> [rst]
  [valid_in] -> Delay4/1
  [rst_in] -> Delay5/1
  Delay4/1 -> [valid]
  Constant7/1 -> AddSub/1
  Logical6/1 -> tap_number/2
  Constant3/1 -> Relational3/2
  element_number/1 -> Delay2/1, Relational3/1
  Logical/1 -> line_number/2
  line_number/1 -> AddSub/2
  Inverter/1 -> Logical3/2, [last_triangle]
  Convert/1 -> Relational1/1
  Relational1/1 -> Inverter/1
  Constant/1 -> Relational/1
  AddSub/1 -> Relational1/2
  tap_number/1 -> Relational/2, Relational4/2, Convert/1
  Gateway Out7/1 -> wr_ctl_debug/5
  Gateway Out4/1 -> wr_ctl_debug/4
  Gateway Out5/1 -> wr_ctl_debug/1
  Gateway Out6/1 -> wr_ctl_debug/2
  Gateway Out8/1 -> wr_ctl_debug/3
  Gateway Out1/1 -> wr_ctl_debug/6
  Gateway Out2/1 -> wr_ctl_debug/7
  [rst_in] -> tap_number/1
  [rst_in] -> line_number/1
  [rst_in] -> element_number/1
  [rst] -> Gateway Out5/1
  [last_triangle] -> Gateway Out4/1
  Constant5/1 -> Relational4/1
  [pos_cnt] -> Gateway Out1/1
  Relational4/1 -> Logical3/1
  Logical3/1 -> [blank_it]
  [blank_it] -> Inverter1/1
  [last_triangle] -> Logical4/1
  Inverter1/1 -> Logical4/2
  Logical4/1 -> Counter2/2
  Counter2/1 -> Mux/3, Gateway Out7/1
  Counter3/1 -> Mux/2
  [rst] -> Counter2/1
  [last_triangle] -> Mux/1
  Mux/1 -> write_addr/1, Gateway Out2/1
  [last_triangle] -> Inverter2/1
  [rst] -> Counter3/1
  Logical5/1 -> Counter3/2
  [valid] -> Logical4/3
  [valid] -> Logical5/1
  Inverter2/1 -> Logical5/2
  [blank_it] -> Inverter3/1
  Inverter3/1 -> Logical7/1
  [valid] -> Logical7/2
  Gateway Out3/1 -> wr_ctl_debug/8
  Logical7/1 -> enable/1, Gateway Out3/1
  Relational3/1 -> posedge1/1
  [valid] -> Gateway Out8/1
  [blank_it] -> Gateway Out6/1

== system r2_b16a4x512f/sys2/xeng/xeng_descramble/x_cast ==
  in : Inport
  Concat : xbsIndex_r4/Concat  num_inputs=8  dbl_ovrd=off  block_type=concat
      settings: block_version=9.2.01
  Convert{,1..7} (8 alike) : xbsIndex_r4/Convert  gui_display_data_type=Fixed-point  arith_type="Signed  (2's comp)"  n_bits=n_bits_out  bin_pt=fix_pnt_pos  float_type=Single  exp_bits=8  fraction_bits=24  quantization=Truncate  overflow=Wrap  en=off  latency=0  dbl_ovrd=off  pipeline=off  block_type=convert
      settings: block_version=10.1.3
  Slice : xbsIndex_r4/Slice  nbits=n_bits_in  boolean_output=off  mode=Lower Bit Location + Width  bit1=0  base1=MSB of Input  bit0=bit_offsets(1)*n_bits_in  base0=LSB of Input  dbl_ovrd=off  block_type=slice
      settings: infoedit="Extracts a given range of bits from each input sample and presents it at the output.  The output type is ordinarily unsigned with binary point at zero, but can be Boolean when the slice is one bit wide.<P><P>Hardware notes: In hardware this block costs nothing."  block_version=10.1.3
  Slice1 : xbsIndex_r4/Slice  nbits=n_bits_in  boolean_output=off  mode=Lower Bit Location + Width  bit1=0  base1=MSB of Input  bit0=bit_offsets(2)*n_bits_in  base0=LSB of Input  dbl_ovrd=off  block_type=slice
      settings: infoedit="Extracts a given range of bits from each input sample and presents it at the output.  The output type is ordinarily unsigned with binary point at zero, but can be Boolean when the slice is one bit wide.<P><P>Hardware notes: In hardware this block costs nothing."  block_version=10.1.3
  Slice2 : xbsIndex_r4/Slice  nbits=n_bits_in  boolean_output=off  mode=Lower Bit Location + Width  bit1=0  base1=MSB of Input  bit0=bit_offsets(3)*n_bits_in  base0=LSB of Input  dbl_ovrd=off  block_type=slice
      settings: infoedit="Extracts a given range of bits from each input sample and presents it at the output.  The output type is ordinarily unsigned with binary point at zero, but can be Boolean when the slice is one bit wide.<P><P>Hardware notes: In hardware this block costs nothing."  block_version=10.1.3
  Slice3 : xbsIndex_r4/Slice  nbits=n_bits_in  boolean_output=off  mode=Lower Bit Location + Width  bit1=0  base1=MSB of Input  bit0=bit_offsets(4)*n_bits_in  base0=LSB of Input  dbl_ovrd=off  block_type=slice
      settings: infoedit="Extracts a given range of bits from each input sample and presents it at the output.  The output type is ordinarily unsigned with binary point at zero, but can be Boolean when the slice is one bit wide.<P><P>Hardware notes: In hardware this block costs nothing."  block_version=10.1.3
  Slice4 : xbsIndex_r4/Slice  nbits=n_bits_in  boolean_output=off  mode=Lower Bit Location + Width  bit1=0  base1=MSB of Input  bit0=bit_offsets(5)*n_bits_in  base0=LSB of Input  dbl_ovrd=off  block_type=slice
      settings: infoedit="Extracts a given range of bits from each input sample and presents it at the output.  The output type is ordinarily unsigned with binary point at zero, but can be Boolean when the slice is one bit wide.<P><P>Hardware notes: In hardware this block costs nothing."  block_version=10.1.3
  Slice5 : xbsIndex_r4/Slice  nbits=n_bits_in  boolean_output=off  mode=Lower Bit Location + Width  bit1=0  base1=MSB of Input  bit0=bit_offsets(6)*n_bits_in  base0=LSB of Input  dbl_ovrd=off  block_type=slice
      settings: infoedit="Extracts a given range of bits from each input sample and presents it at the output.  The output type is ordinarily unsigned with binary point at zero, but can be Boolean when the slice is one bit wide.<P><P>Hardware notes: In hardware this block costs nothing."  block_version=10.1.3
  Slice6 : xbsIndex_r4/Slice  nbits=n_bits_in  boolean_output=off  mode=Lower Bit Location + Width  bit1=0  base1=MSB of Input  bit0=bit_offsets(7)*n_bits_in  base0=LSB of Input  dbl_ovrd=off  block_type=slice
      settings: infoedit="Extracts a given range of bits from each input sample and presents it at the output.  The output type is ordinarily unsigned with binary point at zero, but can be Boolean when the slice is one bit wide.<P><P>Hardware notes: In hardware this block costs nothing."  block_version=10.1.3
  Slice7 : xbsIndex_r4/Slice  nbits=n_bits_in  boolean_output=off  mode=Lower Bit Location + Width  bit1=0  base1=MSB of Input  bit0=bit_offsets(8)*n_bits_in  base0=LSB of Input  dbl_ovrd=off  block_type=slice
      settings: infoedit="Extracts a given range of bits from each input sample and presents it at the output.  The output type is ordinarily unsigned with binary point at zero, but can be Boolean when the slice is one bit wide.<P><P>Hardware notes: In hardware this block costs nothing."  block_version=10.1.3
  force_re{,1,4,6,8,10,12,14} (8 alike) : xbsIndex_r4/Reinterpret  force_arith_type=on  arith_type="Signed  (2's comp)"  force_bin_pt=on  bin_pt=fix_pnt_pos  block_type=reinterpret
      settings: infoedit="Changes signal type without altering the binary representation.   You can changed the signal between signed and unsigned, and relocate the binary point.<P><P>Hardware notes: In hardware this block costs nothing.<P><P>Example:  Suppose the input is 6 bits wide, signed, with 2 fractional bits, and the output is forced to unsigned with 0 fractional bits.  Then an input of -2.0 (1110.00 in binary 2's complement) becomes an output of 56 (111000 in binary)."  block_version=9.1.01
  force_re{2..3,5,7,9,11,13,15} (8 alike) : xbsIndex_r4/Reinterpret  force_arith_type=on  arith_type=Unsigned  force_bin_pt=on  bin_pt=0  block_type=reinterpret
      settings: infoedit="Changes signal type without altering the binary representation.   You can changed the signal between signed and unsigned, and relocate the binary point.<P><P>Hardware notes: In hardware this block costs nothing.<P><P>Example:  Suppose the input is 6 bits wide, signed, with 2 fractional bits, and the output is forced to unsigned with 0 fractional bits.  Then an input of -2.0 (1110.00 in binary 2's complement) becomes an output of 56 (111000 in binary)."  block_version=9.1.01
  out : Outport
  wires:
  force_re15/1 -> Concat/8
  force_re13/1 -> Concat/7
  force_re11/1 -> Concat/6
  force_re9/1 -> Concat/5
  force_re7/1 -> Concat/4
  force_re5/1 -> Concat/3
  Slice7/1 -> force_re14/1
  force_re14/1 -> Convert7/1
  Convert7/1 -> force_re15/1
  Slice6/1 -> force_re12/1
  force_re12/1 -> Convert6/1
  Convert6/1 -> force_re13/1
  Slice5/1 -> force_re10/1
  force_re10/1 -> Convert5/1
  Convert5/1 -> force_re11/1
  Slice4/1 -> force_re8/1
  force_re8/1 -> Convert4/1
  Convert4/1 -> force_re9/1
  Slice3/1 -> force_re6/1
  force_re6/1 -> Convert3/1
  Convert3/1 -> force_re7/1
  Slice2/1 -> force_re4/1
  force_re4/1 -> Convert2/1
  Convert2/1 -> force_re5/1
  force_re3/1 -> Concat/2
  Slice1/1 -> force_re1/1
  Concat/1 -> out/1
  in/1 -> Slice1/1, Slice2/1, Slice3/1, Slice4/1, Slice5/1, Slice7/1, Slice6/1, Slice/1
  Slice/1 -> force_re/1
  force_re1/1 -> Convert1/1
  force_re/1 -> Convert/1
  Convert1/1 -> force_re3/1
  Convert/1 -> force_re2/1
  force_re2/1 -> Concat/1
